simulink model "electric_test"  (R2022b)
settings: Solver=VariableStepAuto  StartTime=0.0  StopTime=1.0  RelTol=1e-3
undefined symbols (not defined in the file or in its folder): D_PI_I, D_PI_KB, D_PI_LOW_LIMIT, D_PI_P, D_PI_UP_LIMIT, Q_PI_I, Q_PI_KB, Q_PI_LOW_LIMIT, Q_PI_P, Q_PI_UP_LIMIT
libraries: simulink x2, slpidlib x2, spsDCVoltageSourceLib x1, spsGroundLib x1, spsPermanentMagnetSynchronousMachineLib x1, spsThreePhaseVIMeasurementLib x1, spsUniversalBridgeLib x1, sps_lib x1
settings Model: Creator=15403  LastModifiedBy=15403

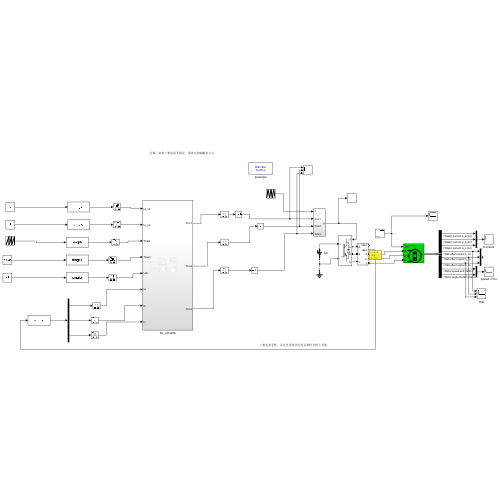
[thumbnail: Simulink's stored preview of the top-level diagram]
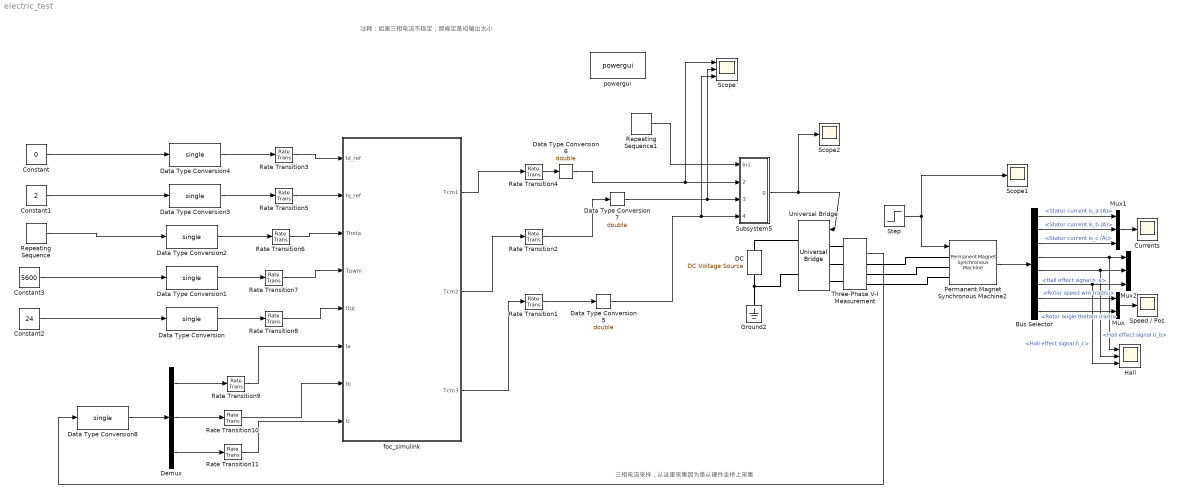
== system electric_test ==
  note: 三相电流采样，从这里采集因为是从硬件全桥上采集
  note: 注释：如果三相电流不稳定，那肯定是IQ输出太小
  Bus Selector : BusSelector  OutputSignals=Stator current is_a (A),Stator current is_b (A),Stator current is_c (A),Hall effect signal h_a,Hall effect signal h_b,Hall effect signal h_c,Rotor speed wm (rad/s),Rotor angle thetam (rad)
  Constant : Constant  Value=0
  Constant1 : Constant  Value=2
  Constant2 : Constant  Value=24
  Constant3 : Constant  Value=5600
  Currents : Scope
  "DC " : spsDCVoltageSourceLib/DC Voltage Source  Amplitude=24  Measurements=None
  Data Type Conversion{,1..4,8} (6 alike) : DataTypeConversion  OutDataTypeStr=single  SaturateOnIntegerOverflow=off  RndMeth=Floor
  Data Type Conversion5 : DataTypeConversion  OutDataTypeStr=double  SaturateOnIntegerOverflow=off  RndMeth=Floor
  Data Type Conversion6 : DataTypeConversion  OutDataTypeStr=double  SaturateOnIntegerOverflow=off  RndMeth=Floor
  Data Type Conversion7 : DataTypeConversion  OutDataTypeStr=double  SaturateOnIntegerOverflow=off  RndMeth=Floor
  Demux : Demux  Outputs=3
  Ground2 : spsGroundLib/Ground  LConnTagsString=a
  Hall : Scope  NumInputPorts=3
  Mux : Mux  Inputs=2
  Mux1 : Mux  Inputs=3
  Mux2 : Mux  Inputs=3
  Permanent Magnet Synchronous Machine2 : spsPermanentMagnetSynchronousMachineLib/Permanent Magnet Synchronous Machine  NbPhases=3  FluxDistribution=Sinusoidal  RotorType=Round  MechanicalLoad=Torque Tm  PresetModel=No  ShowDetailedParameters=on  MeasurementBus=off  Resistance=0.6  Inductance=8.5e-3  dqInductances=[8.5e-3, 8.5e-3]  La=1.4e-3  MachineConstant=Flux linkage established by magnets (V.s)  Flux=0.034182  VoltageCst=6.1999  TorqueCst=0.051273  Flat=120  Mechanical=[1.1e-5,1e-4,1,0.02]  PolePairs=4  InitialConditions=[0,0, 0,0]  InitialConditions5ph=[0 0 0 0 0 0]  RefAngle=Aligned with phase A axis (original Park)  IterativeDiscreteModel=Trapezoidal non iterative  TsBlock=-1  TsPowergui=0
  Rate Transition{1..11} (11 alike) : RateTransition
  Repeating Sequence : simulink/Sources/Repeating Sequence  rep_seq_t=[0 0.1]  rep_seq_y=[0 2 * pi]
  Repeating Sequence1 : simulink/Sources/Repeating Sequence  rep_seq_t=[0 1/15000 2/15000]  rep_seq_y=[0 2800 0]
  Scope : Scope  NumInputPorts=3
  Scope1 : Scope
  Scope2 : Scope
  Speed / Pos : Scope
  Step : Step  Time=0  After=0  SampleTime=0
  Subsystem5 : Subsystem
  Three-Phase V-I Measurement : spsThreePhaseVIMeasurementLib/Three-Phase V-I Measurement  VoltageMeasurement=phase-to-ground  SetLabelV=off  LabelV=Vabc  Vpu=off  VpuLL=off  CurrentMeasurement=yes  SetLabelI=off  LabelI=Iabc  Ipu=off  Pbase=100e6  Vbase=500e3  OutputType=Complex  PhasorSimulation=off  PSBequivalent=0
  Universal Bridge : spsUniversalBridgeLib/Universal Bridge  Arms=3  SnubberResistance=1e5  SnubberCapacitance=inf  Device=IGBT / Diodes  Ron=1e-3  Lon=0  ForwardVoltages="[  0  0  ]"  ForwardVoltage=0  GTOparameters=[ 10e-6 , 20e-6 ]  IGBTparameters=[ 1e-6 , 2e-6 ]  Measurements=None  Measurements_2=None  converterType=Rectifier
  foc_simulink : Subsystem
  powergui : sps_lib/powergui  Priority=1  SimulationMode=Discrete  SampleTime=0.000001  frequency=60  Iterations=50  frequencyindice=0  Pbase=100e6  ErrMax=1e-4  UnitsV=kV  UnitsW=MW  buscounter=0  FunctionMessages=off  echomessages=off  EnableUseOfTLC=off  CurrentSourceSwitches=off  DisableSnubberDevices=off  DisableRonSwitches=off  DisableVfSwitches=off  DisplayEquations=off  AutomaticDiscreteSolvers=off  SolverType=Tustin/Backward Euler (TBE)  Interpol=off  ExternalGateDelay=off  methode=off  Ts=100  x0status=blocks  SPID=on  SwTol=0  HookPort=off  NonlinearTolerance=1e-4  nMaxIteration=100  ContinueOnMaxIteration=off  RestoreLinks=warning  ResistiveCurrentMeasurement=off  Frange=[0:2:500]  Ylog=off  Xlog=on  ShowGrid=off  save=off  variable=ZData  structure=0  ZoomFFT=off  StartTime=0.0  cycles=1  DisplayStyle=1  fundamental=60  FreqAxis=off  MaxFrequency=1000  frequencyindicesteady=1  RmsSteady=1  display=off
  wires:
  Demux/3 -> Rate Transition11/1
  Data Type Conversion/1 -> Rate Transition8/1
  Repeating Sequence1/1 -> Subsystem5/1(In1)
  foc_simulink/3(Tcm3) -> Rate Transition1/1
  Mux/1 -> Speed / Pos/1
  foc_simulink/1(Tcm1) -> Rate Transition4/1
  Mux1/1 -> Currents/1
  Step/1 -> Permanent Magnet Synchronous Machine2/1, Scope1/1
  Rate Transition6/1 -> foc_simulink/3(Theta)
  Rate Transition11/1 -> foc_simulink/8(Ic)
  Data Type Conversion5/1 -> Subsystem5/4(Tcm3), Scope/3
  Constant1/1 -> Data Type Conversion3/1
  Rate Transition2/1 -> Data Type Conversion7/1
  Three-Phase V-I Measurement/2 -> Data Type Conversion8/1
  Constant2/1 -> Data Type Conversion/1
  Rate Transition8/1 -> foc_simulink/5(Udc)
  Permanent Magnet Synchronous Machine2/1 -> Bus Selector/1
  Bus Selector/8 -> Mux/2  "<Rotor angle thetam (rad)>"
  Rate Transition9/1 -> foc_simulink/6(Ia)
  Repeating Sequence/1 -> Data Type Conversion2/1
  Constant/1 -> Data Type Conversion4/1
  Data Type Conversion4/1 -> Rate Transition3/1
  Rate Transition4/1 -> Data Type Conversion6/1
  Rate Transition1/1 -> Data Type Conversion5/1
  Bus Selector/5 -> Mux2/2, Hall/2  "<Hall effect signal h_b>"
  Data Type Conversion6/1 -> Scope/1, Subsystem5/2(Tcm1)
  Bus Selector/3 -> Mux1/3  "<Stator current is_c (A)>"
  foc_simulink/2(Tcm2) -> Rate Transition2/1
  Constant3/1 -> Data Type Conversion1/1
  Subsystem5/1(g) -> Scope2/1, Universal Bridge/1
  Data Type Conversion1/1 -> Rate Transition7/1
  Bus Selector/7 -> Mux/1  "<Rotor speed wm (rad/s)>"
  Bus Selector/1 -> Mux1/1  "<Stator current is_a (A)>"
  Demux/1 -> Rate Transition9/1
  Rate Transition7/1 -> foc_simulink/4(Tpwm)
  Data Type Conversion7/1 -> Scope/2, Subsystem5/3(Tcm2)
  Bus Selector/4 -> Hall/1, Mux2/1  "<Hall effect signal h_a>"
  Data Type Conversion2/1 -> Rate Transition6/1
  Bus Selector/2 -> Mux1/2  "<Stator current is_b (A)>"
  Demux/2 -> Rate Transition10/1
  Rate Transition5/1 -> foc_simulink/2(Iq_ref)
  Bus Selector/6 -> Mux2/3, Hall/3  "<Hall effect signal h_c>"
  Data Type Conversion8/1 -> Demux/1
  Rate Transition3/1 -> foc_simulink/1(Id_ref)
  Data Type Conversion3/1 -> Rate Transition5/1
  Rate Transition10/1 -> foc_simulink/7(Ib)
  connections:
  Universal Bridge/RConn2 -- Ground2/LConn1 -- "DC "/LConn1
  Permanent Magnet Synchronous Machine2/LConn1 -- Three-Phase V-I Measurement/RConn1
  Universal Bridge/LConn3 -- Three-Phase V-I Measurement/LConn3
  Universal Bridge/LConn1 -- Three-Phase V-I Measurement/LConn1
  Permanent Magnet Synchronous Machine2/LConn3 -- Three-Phase V-I Measurement/RConn3
  Universal Bridge/LConn2 -- Three-Phase V-I Measurement/LConn2
  Permanent Magnet Synchronous Machine2/LConn2 -- Three-Phase V-I Measurement/RConn2
  "DC "/RConn1 -- Universal Bridge/RConn1

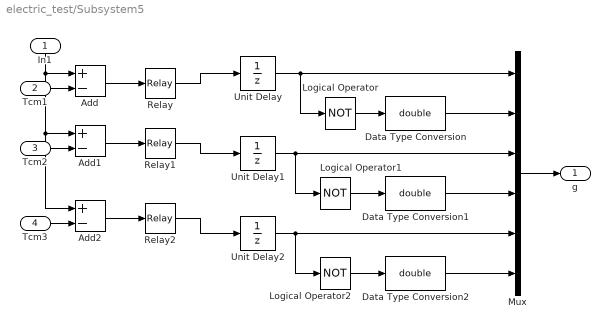
== system electric_test/Subsystem5 ==
  In1 : Inport
  Tcm1 : Inport  Port=2
  Tcm2 : Inport  Port=3
  Tcm3 : Inport  Port=4
  Add : Sum  Inputs=+-
  Add1 : Sum  Inputs=+-
  Add2 : Sum  Inputs=+-
  Data Type Conversion : DataTypeConversion  OutDataTypeStr=double  SaturateOnIntegerOverflow=off  RndMeth=Floor
  Data Type Conversion1 : DataTypeConversion  OutDataTypeStr=double  SaturateOnIntegerOverflow=off  RndMeth=Floor
  Data Type Conversion2 : DataTypeConversion  OutDataTypeStr=double  SaturateOnIntegerOverflow=off  RndMeth=Floor
  Logical Operator : Logic  Operator=NOT  AllPortsSameDT=off  OutDataTypeStr=boolean
  Logical Operator1 : Logic  Operator=NOT  AllPortsSameDT=off  OutDataTypeStr=boolean
  Logical Operator2 : Logic  Operator=NOT  AllPortsSameDT=off  OutDataTypeStr=boolean
  Mux : Mux  Inputs=6
  Relay : Relay  OffSwitchValue=-eps
  Relay1 : Relay  OffSwitchValue=-eps
  Relay2 : Relay  OffSwitchValue=-eps
  Unit Delay : UnitDelay  SampleTime=-1  HasFrameUpgradeWarning=on
  Unit Delay1 : UnitDelay  SampleTime=-1  HasFrameUpgradeWarning=on
  Unit Delay2 : UnitDelay  SampleTime=-1  HasFrameUpgradeWarning=on
  g : Outport  VectorParamsAs1DForOutWhenUnconnected=off
  wires:
  Tcm3/1 -> Add2/2
  Tcm2/1 -> Add1/2
  Tcm1/1 -> Add/2
  Relay2/1 -> Unit Delay2/1
  Relay1/1 -> Unit Delay1/1
  Relay/1 -> Unit Delay/1
  Unit Delay2/1 -> Mux/5, Logical Operator2/1
  Unit Delay1/1 -> Mux/3, Logical Operator1/1
  Unit Delay/1 -> Logical Operator/1, Mux/1
  Mux/1 -> g/1
  Data Type Conversion/1 -> Mux/2
  Data Type Conversion1/1 -> Mux/4
  Data Type Conversion2/1 -> Mux/6
  Logical Operator2/1 -> Data Type Conversion2/1
  Logical Operator1/1 -> Data Type Conversion1/1
  Logical Operator/1 -> Data Type Conversion/1
  Add1/1 -> Relay1/1
  Add2/1 -> Relay2/1
  Add/1 -> Relay/1
  In1/1 -> Add/1, Add2/1, Add1/1

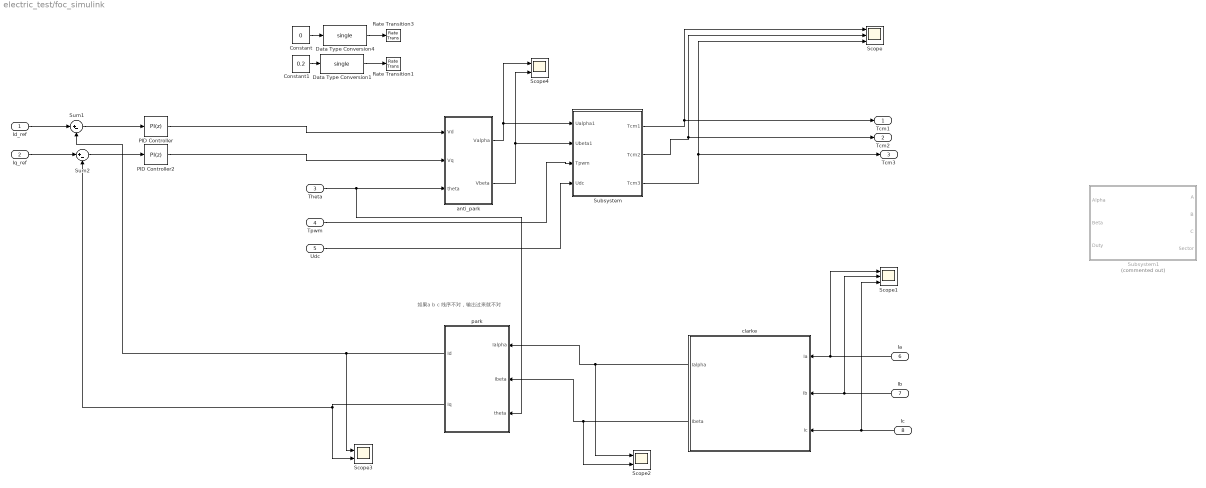
== system electric_test/foc_simulink ==
  note: 如果a b c 线序不对，输出过来就不对
  Id_ref : Inport
  Iq_ref : Inport  Port=2
  Theta : Inport  Port=3
  Tpwm : Inport  Port=4
  Udc : Inport  Port=5
  Ia : Inport  Port=6
  Ib : Inport  Port=7
  Ic : Inport  Port=8
  Constant : Constant  Value=0
  Constant1 : Constant  Value=0.2
  Data Type Conversion1 : DataTypeConversion  OutDataTypeStr=single  SaturateOnIntegerOverflow=off  RndMeth=Floor
  Data Type Conversion4 : DataTypeConversion  OutDataTypeStr=single  SaturateOnIntegerOverflow=off  RndMeth=Floor
  PID Controller : slpidlib/PID Controller  Controller=PI  Form=Parallel  TimeDomain=Discrete-time  UseExternalTs=off  SampleTime=-1  IntegratorMethod=Forward Euler  FilterMethod=Forward Euler  ControllerParametersSource=internal  P=D_PI_P  I=D_PI_I  UseKiTs=off  D=0  N=100  UseFilter=on  TunerSelectOption=Transfer Function Based (PID Tuner App)  InitialConditionSource=internal  InitialConditionForIntegrator=0  InitialConditionForFilter=0  DifferentiatorICPrevScaledInput=0  ExternalReset=none  TrackingMode=off  Kt=1  LimitOutput=on  SatLimitsSource=internal  UpperSaturationLimit=D_PI_UP_LIMIT  LowerSaturationLimit=D_PI_LOW_LIMIT  LinearizeAsGain=off  AntiWindupMode=back-calculation  Kb=D_PI_KB  LimitIntegrator=off  UpperIntegratorSaturationLimit=inf  LowerIntegratorSaturationLimit=-inf  PGainOutDataTypeStr=single  PProdOutDataTypeStr=single  POutMin=[]  POutMax=[]  IGainOutDataTypeStr=single  IProdOutDataTypeStr=single  IOutMin=[]  IOutMax=[]  DOutMin=[]  DOutMax=[]  NOutMin=[]  NOutMax=[]  SumOutDataTypeStr=single  SumOutMin=[]  SumOutMax=[]  SaturationOutDataTypeStr=single  SaturationOutMin=[]  SaturationOutMax=[]  PParamMin=[]  PParamMax=[]  IParamMin=[]  IParamMax=[]  DParamMin=[]  DParamMax=[]  NParamMin=[]  NParamMax=[]  KbParamMin=[]  KbParamMax=[]  KtParamMin=[]  KtParamMax=[]  KbOutMin=[]  KbOutMax=[]  KtOutMin=[]  KtOutMax=[]  IntegratorOutMin=[]  IntegratorOutMax=[]  FilterOutMin=[]  FilterOutMax=[]  SumI1OutMin=[]  SumI1OutMax=[]  SumI2OutMin=[]  SumI2OutMax=[]  SumI3OutMin=[]  SumI3OutMax=[]  SumI4OutMin=[]  SumI4OutMax=[]  SumDOutMin=[]  SumDOutMax=[]  DifferentiatorOutMin=[]  DifferentiatorOutMax=[]  FilterDiffOutCoefMin=[]  FilterDiffOutCoefMax=[]  ReciprocalOutMin=[]  ReciprocalOutMax=[]  SumDenOutMin=[]  SumDenOutMax=[]  SumNumOutMin=[]  SumNumOutMax=[]  DivideOutMin=[]  DivideOutMax=[]  UdiffTsProdOutMin=[]  UdiffTsProdOutMax=[]  NTsProdOutMin=[]  NTsProdOutMax=[]  UintegralTsProdOutMin=[]  UintegralTsProdOutMax=[]  UngainTsProdOutMin=[]  UngainTsProdOutMax=[]  ClampingZeroOutDataTypeStr=Inherit: Inherit via back propagation  ClampingZeroOutMin=[]  ClampingZeroOutMax=[]  FilterDenConstantOutDataTypeStr=Inherit: Inherit via back propagation  FilterDenConstantOutMin=[]  FilterDenConstantOutMax=[]  PCopyOutDataTypeStr=Inherit: Inherit via back propagation  PCopyOutMin=[]  PCopyOutMax=[]  NCopyOutDataTypeStr=Inherit: Inherit via back propagation  NCopyOutMin=[]  NCopyOutMax=[]  IntegratorContinuousStateAttributes=''  IntegratorStateIdentifier=di  IntegratorStateMustResolveToSignalObject=off  IntegratorRTWStateStorageClass=Auto  FilterContinuousStateAttributes=''  FilterStateMustResolveToSignalObject=off  FilterRTWStateStorageClass=Auto  ParallelPVariant=InternalParameters  IdealPVariant=Disabled  IVariant=InternalParameters  DVariant=Disabled  IntegratorVariant=Discrete  SatVariant=Enabled  AWVariant=BackCalculation  PCopyVariant=Disabled  TRVariant=Disabled  FdbkBlocksVariant=Forward  IdealPFdbkVariant=Disabled  SatFdbkVariant=Disabled  DerivativeFilterVariant=Disabled  NVariant=Disabled  NCopyVariant=Disabled_SignalSpec  FilterICVariant=Disabled  IntegratorICVariant=InternalICs  ExternalResetVariant=Disabled  TRSumVariant=Passthrough  SumFdbkVariant=Disabled  SumVariant=Sum_PI  TsampFilterVariant=InternalTs  TsampNgainVariant=Passthrough  TsampIntegralVariant=Passthrough  ExternalSaturationOutDataTypeStr=Inherit: Same as second input
  PID Controller2 : slpidlib/PID Controller  Controller=PI  Form=Parallel  TimeDomain=Discrete-time  UseExternalTs=off  SampleTime=-1  IntegratorMethod=Forward Euler  FilterMethod=Forward Euler  ControllerParametersSource=internal  P=Q_PI_P  I=Q_PI_I  UseKiTs=off  D=0  N=100  UseFilter=on  TunerSelectOption=Transfer Function Based (PID Tuner App)  InitialConditionSource=internal  InitialConditionForIntegrator=0  InitialConditionForFilter=0  DifferentiatorICPrevScaledInput=0  ExternalReset=none  TrackingMode=off  Kt=1  LimitOutput=on  SatLimitsSource=internal  UpperSaturationLimit=Q_PI_UP_LIMIT  LowerSaturationLimit=Q_PI_LOW_LIMIT  LinearizeAsGain=off  AntiWindupMode=back-calculation  Kb=Q_PI_KB  LimitIntegrator=off  UpperIntegratorSaturationLimit=inf  LowerIntegratorSaturationLimit=-inf  PGainOutDataTypeStr=single  PProdOutDataTypeStr=single  POutMin=[]  POutMax=[]  IGainOutDataTypeStr=single  IProdOutDataTypeStr=single  IOutMin=[]  IOutMax=[]  DOutMin=[]  DOutMax=[]  NOutMin=[]  NOutMax=[]  SumOutDataTypeStr=single  SumOutMin=[]  SumOutMax=[]  SaturationOutDataTypeStr=single  SaturationOutMin=[]  SaturationOutMax=[]  PParamMin=[]  PParamMax=[]  IParamMin=[]  IParamMax=[]  DParamMin=[]  DParamMax=[]  NParamMin=[]  NParamMax=[]  KbParamMin=[]  KbParamMax=[]  KtParamMin=[]  KtParamMax=[]  KbOutMin=[]  KbOutMax=[]  KtOutMin=[]  KtOutMax=[]  IntegratorOutMin=[]  IntegratorOutMax=[]  FilterOutMin=[]  FilterOutMax=[]  SumI1OutMin=[]  SumI1OutMax=[]  SumI2OutMin=[]  SumI2OutMax=[]  SumI3OutMin=[]  SumI3OutMax=[]  SumI4OutMin=[]  SumI4OutMax=[]  SumDOutMin=[]  SumDOutMax=[]  DifferentiatorOutMin=[]  DifferentiatorOutMax=[]  FilterDiffOutCoefMin=[]  FilterDiffOutCoefMax=[]  ReciprocalOutMin=[]  ReciprocalOutMax=[]  SumDenOutMin=[]  SumDenOutMax=[]  SumNumOutMin=[]  SumNumOutMax=[]  DivideOutMin=[]  DivideOutMax=[]  UdiffTsProdOutMin=[]  UdiffTsProdOutMax=[]  NTsProdOutMin=[]  NTsProdOutMax=[]  UintegralTsProdOutMin=[]  UintegralTsProdOutMax=[]  UngainTsProdOutMin=[]  UngainTsProdOutMax=[]  ClampingZeroOutDataTypeStr=Inherit: Inherit via back propagation  ClampingZeroOutMin=[]  ClampingZeroOutMax=[]  FilterDenConstantOutDataTypeStr=Inherit: Inherit via back propagation  FilterDenConstantOutMin=[]  FilterDenConstantOutMax=[]  PCopyOutDataTypeStr=Inherit: Inherit via back propagation  PCopyOutMin=[]  PCopyOutMax=[]  NCopyOutDataTypeStr=Inherit: Inherit via back propagation  NCopyOutMin=[]  NCopyOutMax=[]  IntegratorContinuousStateAttributes=''  IntegratorStateIdentifier=qi  IntegratorStateMustResolveToSignalObject=off  IntegratorRTWStateStorageClass=Auto  FilterContinuousStateAttributes=''  FilterStateMustResolveToSignalObject=off  FilterRTWStateStorageClass=Auto  ParallelPVariant=InternalParameters  IdealPVariant=Disabled  IVariant=InternalParameters  DVariant=Disabled  IntegratorVariant=Discrete  SatVariant=Enabled  AWVariant=BackCalculation  PCopyVariant=Disabled  TRVariant=Disabled  FdbkBlocksVariant=Forward  IdealPFdbkVariant=Disabled  SatFdbkVariant=Disabled  DerivativeFilterVariant=Disabled  NVariant=Disabled  NCopyVariant=Disabled_SignalSpec  FilterICVariant=Disabled  IntegratorICVariant=InternalICs  ExternalResetVariant=Disabled  TRSumVariant=Passthrough  SumFdbkVariant=Disabled  SumVariant=Sum_PI  TsampFilterVariant=InternalTs  TsampNgainVariant=Passthrough  TsampIntegralVariant=Passthrough  ExternalSaturationOutDataTypeStr=Inherit: Same as second input
  Rate Transition1 : RateTransition
  Rate Transition3 : RateTransition
  Scope : Scope  NumInputPorts=3
  Scope1 : Scope  NumInputPorts=3
  Scope2 : Scope  NumInputPorts=2
  Scope3 : Scope  NumInputPorts=2
  Scope4 : Scope  NumInputPorts=2
  Subsystem : Subsystem
  Subsystem1 : Subsystem  Commented=on
  Sum1 : Sum  Inputs=|+-
  Sum2 : Sum  Inputs=|+-
  anti_park : Subsystem
  clarke : Subsystem
  park : Subsystem
  Tcm1 : Outport
  Tcm2 : Outport  Port=2
  Tcm3 : Outport  Port=3
  wires:
  Udc/1 -> Subsystem/4(Udc)
  Tpwm/1 -> Subsystem/3(Tpwm)
  Subsystem/3(Tcm3) -> Tcm3/1, Scope/3
  anti_park/2(Vbeta) -> Subsystem/2(Ubeta1), Scope4/2
  Subsystem/1(Tcm1) -> Tcm1/1, Scope/1
  Subsystem/2(Tcm2) -> Tcm2/1, Scope/2
  anti_park/1(Valpha) -> Subsystem/1(Ualpha1), Scope4/1
  clarke/2(Ibeta) -> Scope2/2, park/2(Ibeta)
  clarke/1(Ialpha) -> Scope2/1, park/1(Ialpha)
  Ia/1 -> Scope1/1, clarke/1(Ia)
  Ib/1 -> Scope1/2, clarke/2(Ib)
  Ic/1 -> Scope1/3, clarke/3(Ic)
  park/1(Id) -> Sum1/2, Scope3/1
  park/2(Iq) -> Sum2/2, Scope3/2
  Id_ref/1 -> Sum1/1
  Sum1/1 -> PID Controller/1
  Iq_ref/1 -> Sum2/1
  Sum2/1 -> PID Controller2/1
  Theta/1 -> park/3(theta), anti_park/3(theta)
  PID Controller/1 -> anti_park/1(Vd)
  PID Controller2/1 -> anti_park/2(Vq)
  Data Type Conversion1/1 -> Rate Transition1/1
  Data Type Conversion4/1 -> Rate Transition3/1
  Constant/1 -> Data Type Conversion4/1
  Constant1/1 -> Data Type Conversion1/1

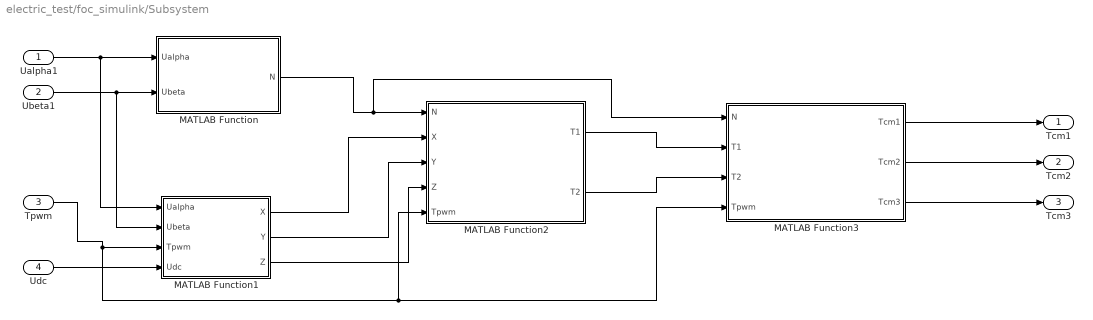
== system electric_test/foc_simulink/Subsystem ==
  Ualpha1 : Inport
  Ubeta1 : Inport  Port=2
  Tpwm : Inport  Port=3
  Udc : Inport  Port=4
  MATLAB Function : MATLAB Function  TreatAsAtomicUnit=on
  MATLAB Function1 : MATLAB Function  TreatAsAtomicUnit=on
  MATLAB Function2 : MATLAB Function  TreatAsAtomicUnit=on
  MATLAB Function3 : MATLAB Function  TreatAsAtomicUnit=on
  Tcm1 : Outport
  Tcm2 : Outport  Port=2
  Tcm3 : Outport  Port=3
  wires:
  MATLAB Function3/2(Tcm2) -> Tcm2/1
  Tpwm/1 -> MATLAB Function3/4(Tpwm), MATLAB Function2/5(Tpwm), MATLAB Function1/3(Tpwm)
  MATLAB Function/1(N) -> MATLAB Function3/1(N), MATLAB Function2/1(N)
  Udc/1 -> MATLAB Function1/4(Udc)
  MATLAB Function3/3(Tcm3) -> Tcm3/1
  MATLAB Function2/1(T1) -> MATLAB Function3/2(T1)
  Ualpha1/1 -> MATLAB Function1/1(Ualpha), MATLAB Function/1(Ualpha)
  MATLAB Function2/2(T2) -> MATLAB Function3/3(T2)
  Ubeta1/1 -> MATLAB Function1/2(Ubeta), MATLAB Function/2(Ubeta)
  MATLAB Function3/1(Tcm1) -> Tcm1/1
  MATLAB Function1/1(X) -> MATLAB Function2/2(X)
  MATLAB Function1/3(Z) -> MATLAB Function2/4(Z)
  MATLAB Function1/2(Y) -> MATLAB Function2/3(Y)

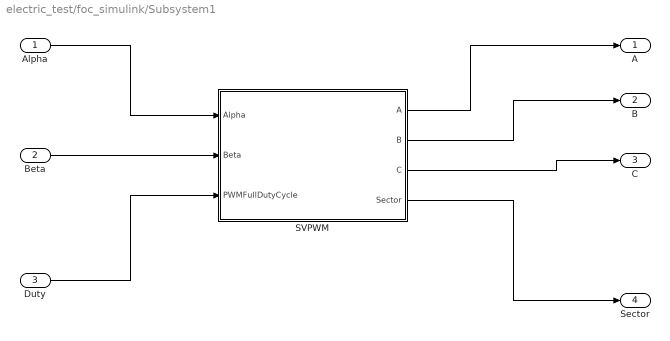
== system electric_test/foc_simulink/Subsystem1 ==
  Alpha : Inport
  Beta : Inport  Port=2
  Duty : Inport  Port=3
  SVPWM : MATLAB Function  TreatAsAtomicUnit=on
  A : Outport
  B : Outport  Port=2
  C : Outport  Port=3
  Sector : Outport  Port=4
  wires:
  SVPWM/1(A) -> A/1
  Duty/1 -> SVPWM/3(PWMFullDutyCycle)
  Alpha/1 -> SVPWM/1(Alpha)
  Beta/1 -> SVPWM/2(Beta)
  SVPWM/3(C) -> C/1
  SVPWM/4(Sector) -> Sector/1
  SVPWM/2(B) -> B/1

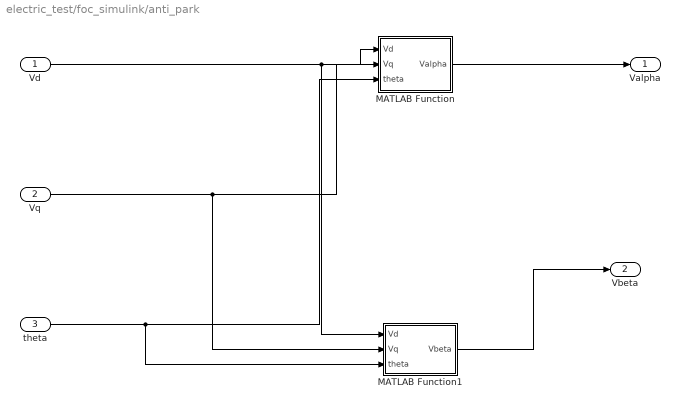
== system electric_test/foc_simulink/anti_park ==
  Vd : Inport
  Vq : Inport  Port=2
  theta : Inport  Port=3
  MATLAB Function : MATLAB Function  TreatAsAtomicUnit=on
  MATLAB Function1 : MATLAB Function  TreatAsAtomicUnit=on
  Valpha : Outport
  Vbeta : Outport  Port=2
  wires:
  MATLAB Function/1(Valpha) -> Valpha/1
  MATLAB Function1/1(Vbeta) -> Vbeta/1
  Vd/1 -> MATLAB Function/1(Vd), MATLAB Function1/1(Vd)
  Vq/1 -> MATLAB Function/2(Vq), MATLAB Function1/2(Vq)
  theta/1 -> MATLAB Function/3(theta), MATLAB Function1/3(theta)

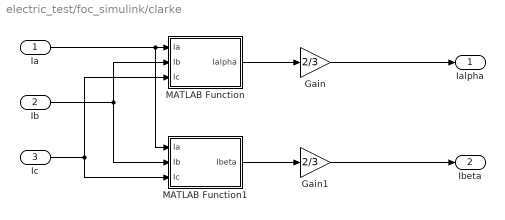
== system electric_test/foc_simulink/clarke ==
  Ia : Inport
  Ib : Inport  Port=2
  Ic : Inport  Port=3
  Gain : Gain  Gain=2/3  OutDataTypeStr=single
  Gain1 : Gain  Gain=2/3  OutDataTypeStr=single
  MATLAB Function : MATLAB Function  TreatAsAtomicUnit=on
  MATLAB Function1 : MATLAB Function  TreatAsAtomicUnit=on
  Ialpha : Outport
  Ibeta : Outport  Port=2
  wires:
  Ia/1 -> MATLAB Function1/1(Ia), MATLAB Function/1(Ia)
  MATLAB Function/1(Ialpha) -> Gain/1
  Gain1/1 -> Ibeta/1
  Ib/1 -> MATLAB Function1/2(Ib), MATLAB Function/2(Ib)
  Ic/1 -> MATLAB Function/3(Ic), MATLAB Function1/3(Ic)
  MATLAB Function1/1(Ibeta) -> Gain1/1
  Gain/1 -> Ialpha/1

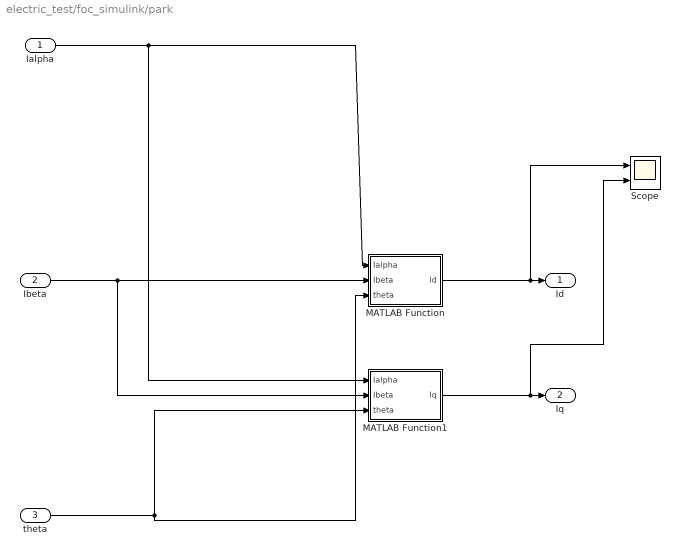
== system electric_test/foc_simulink/park ==
  Ialpha : Inport
  Ibeta : Inport  Port=2
  theta : Inport  Port=3
  MATLAB Function : MATLAB Function  TreatAsAtomicUnit=on
  MATLAB Function1 : MATLAB Function  TreatAsAtomicUnit=on
  Scope : Scope  NumInputPorts=2
  Id : Outport
  Iq : Outport  Port=2
  wires:
  theta/1 -> MATLAB Function/3(theta), MATLAB Function1/3(theta)
  Ibeta/1 -> MATLAB Function/2(Ibeta), MATLAB Function1/2(Ibeta)
  MATLAB Function1/1(Iq) -> Scope/2, Iq/1
  MATLAB Function/1(Id) -> Scope/1, Id/1
  Ialpha/1 -> MATLAB Function/1(Ialpha), MATLAB Function1/1(Ialpha)

== matlab function electric_test/foc_simulink/park/MATLAB Function ==
  data: Ialpha input; Id output; Ibeta input; theta input
function Id = fcn(Ialpha, Ibeta, theta)

Id = Ialpha * cos(theta) + Ibeta * sin(theta);

== matlab function electric_test/foc_simulink/park/MATLAB Function1 ==
  data: Ialpha input; Iq output; Ibeta input; theta input
function Iq = fcn(Ialpha, Ibeta, theta)
Iq = -Ialpha * sin(theta) + Ibeta * cos(theta);

== matlab function electric_test/foc_simulink/anti_park/MATLAB Function1 ==
  data: Vd input; Vbeta output; Vq input; theta input
function Vbeta = fcn(Vd, Vq, theta)

Vbeta = Vd * sin(theta) + Vq * cos(theta);

== matlab function electric_test/foc_simulink/anti_park/MATLAB Function ==
  data: Vd input; Valpha output; Vq input; theta input
function Valpha = fcn(Vd, Vq, theta)

Valpha = Vd * cos(theta) - Vq * sin(theta);

== matlab function electric_test/foc_simulink/Subsystem1/SVPWM ==
  data: Alpha input; A output; B output; C output; Sector output; Beta input; PWMFullDutyCycle input
function [A, B, C, Sector] = fcn(Alpha, Beta, PWMFullDutyCycle)

% 初始化变量
A = single(0);
B = single(0);
C = single(0);                                  
Sector = 0;
ONE_BY_SQRT3 = tand(30);
TWO_BY_SQRT3 = (2.0 * 0.57735026919);

% 扇区判断
if Beta >= 0.0
    if Alpha >= 0.0
        if (ONE_BY_SQRT3 * Beta) > Alpha
                Sector = 2;
        else
            Sector = 1;
        end
    else
        if -ONE_BY_SQRT3 * Beta > Alpha
            Sector = 3;
        else
            Sector = 2;
        end
    end
else
    if Alpha >= 0.0
        if -ONE_BY_SQRT3 * Beta > Alpha
            Sector = 5;
        else
            Sector = 6;
        end

    else
        if ONE_BY_SQRT3 * Beta > Alpha
            Sector = 4;
        else
            Sector = 5;
        end
    end
end


switch Sector
    case 1
        t1 = (Alpha - ONE_BY_SQRT3 * Beta) * PWMFullDutyCycle;
        t2 = (TWO_BY_SQRT3 * Beta) * PWMFullDutyCycle;

        A = (PWMFullDutyCycle + t1 + t2) / 2;
        B = A - t1;
        C = B - t2;
    case 2
		t2 = (Alpha + ONE_BY_SQRT3 * Beta) * PWMFullDutyCycle;
		t3 = (-Alpha + ONE_BY_SQRT3 * Beta) * PWMFullDutyCycle;

		B = (PWMFullDutyCycle + t2 + t3) / 2;
		A = B - t3;
		C = A - t2;
        
    case 3
       t3 = (TWO_BY_SQRT3 * Beta) * PWMFullDutyCycle;
		t4 = (-Alpha - ONE_BY_SQRT3 * Beta) * PWMFullDutyCycle;

		B = (PWMFullDutyCycle + t3 + t4) / 2;
		C = B - t3;
		A = C - t4;

    case 4
		t4 = (-Alpha + ONE_BY_SQRT3 * Beta) * PWMFullDutyCycle;
		t5 = (-TWO_BY_SQRT3 * Beta) * PWMFullDutyCycle;

		C = (PWMFullDutyCycle + t4 + t5) / 2;
		B = C - t5;
		A = B - t4;
    case 5
        t5 = (-Alpha - ONE_BY_SQRT3 * Beta) * PWMFullDutyCycle;
		t6 = (Alpha - ONE_BY_SQRT3 * Beta) * PWMFullDutyCycle;

		C = (PWMFullDutyCycle + t5 + t6) / 2;
		A = C - t5;
		B = A - t6;

    case 6
		t6 = (-TWO_BY_SQRT3 * Beta) * PWMFullDutyCycle;
		t1 = (Alpha + ONE_BY_SQRT3 * Beta) * PWMFullDutyCycle;

		A = (PWMFullDutyCycle + t6 + t1) / 2;
		C = A - t1;
		B = C - t6;
end

== matlab function electric_test/foc_simulink/Subsystem/MATLAB Function ==
  data: Ualpha input; N output; Ubeta input
function N = fcn(Ualpha, Ubeta)

U1 = Ubeta;
U2 = sqrt(3) * Ualpha - Ubeta;
U3 = -sqrt(3) * Ualpha - Ubeta;
A = 0;
B = 0;
C = 0;

if U1 > 0
    A = 1;
else
    A = 0;
end

if U2 > 0
    B = 1;
else
    B = 0;
end

if U3 > 0
    C = 1;
else
    C = 0;
end

N = A + 2 * B + 4 * C;

== matlab function electric_test/foc_simulink/Subsystem/MATLAB Function1 ==
  data: Ualpha input; Ubeta input; Tpwm input; Udc input; X output; Y output; Z output
function [X, Y, Z] = fcn(Ualpha, Ubeta, Tpwm, Udc)

X = sqrt(3) * Tpwm * Ubeta / Udc;
Y = sqrt(3) * Tpwm / Udc * (sqrt(3) / 2 * Ualpha + 1 / 2 * Ubeta);
Z = sqrt(3) * Tpwm / Udc * (-sqrt(3) / 2 * Ualpha + 1 / 2 * Ubeta);

== matlab function electric_test/foc_simulink/Subsystem/MATLAB Function2 ==
  data: N input; T1 output; X input; Y input; Z input; Tpwm input; T2 output
function [T1, T2] = fcn(N, X, Y, Z, Tpwm)

T1 = single(0);
T2 = single(0);

if N == 1
    T1 = Z;
    T2 = Y;
elseif N == 2
    T1 = Y;
    T2 = -X;
elseif N == 3
    T1 = -Z;
    T2 = X;
elseif N == 4
    T1 = -X;
    T2 = Z;
elseif N == 5
    T1 = X;
    T2 = -Y;
elseif N == 6
    T1 = -Y;
    T2 = -Z;
end

== matlab function electric_test/foc_simulink/Subsystem/MATLAB Function3 ==
  data: N input; Tcm1 output; T1 input; T2 input; Tpwm input; Tcm2 output; Tcm3 output
function [Tcm1, Tcm2, Tcm3] = fcn(N, T1, T2, Tpwm)

Tcm1 = single(0);
Tcm2 = single(0);
Tcm3 = single(0);


if N == 1
    Tcm1 = (Tpwm + T1 - T2) / 4;
    Tcm2 = (Tpwm - T1 - T2) / 4;
    Tcm3 = (Tpwm + T1 + T2) / 4;
elseif N == 2
    Tcm1 = (Tpwm - T1 - T2) / 4;
    Tcm2 = (Tpwm + T1 + T2) / 4;
    Tcm3 = (Tpwm + T1 - T2) / 4;
elseif N == 3
    Tcm1 = (Tpwm - T1 - T2) / 4;
    Tcm2 = (Tpwm + T1 - T2) / 4;
    Tcm3 = (Tpwm + T1 + T2) / 4;
elseif N == 4
    Tcm1 = (Tpwm + T1 + T2) / 4;
    Tcm2 = (Tpwm + T1 - T2) / 4;
    Tcm3 = (Tpwm - T1 - T2) / 4;
elseif N == 5
    Tcm1 = (Tpwm + T1 + T2) / 4;
    Tcm2 = (Tpwm - T1 - T2) / 4;
    Tcm3 = (Tpwm + T1 - T2) / 4;
elseif N == 6
    Tcm1 = (Tpwm + T1 - T2) / 4;
    Tcm2 = (Tpwm + T1 + T2) / 4;
    Tcm3 = (Tpwm - T1 - T2) / 4;
end

== matlab function electric_test/foc_simulink/clarke/MATLAB Function ==
  data: Ia input; Ialpha output; Ib input; Ic input
function Ialpha = fcn(Ia, Ib, Ic)

Ialpha = 3/2 * Ia;

== matlab function electric_test/foc_simulink/clarke/MATLAB Function1 ==
  data: Ia input; Ibeta output; Ib input; Ic input
function Ibeta = fcn( Ia, Ib, Ic)

Ibeta = sqrt(3)/2 * (Ia + 2 * Ib);
